simulink model "Sensors"  (R2026a)
settings: Solver=FixedStepAuto
values from neighbouring files (symbols this model uses):
  SNS = loadSensorParameters()    [ch7_main.m]    (also in loadSensorParameters.m = struct())
undefined symbols (not defined in the file or in its folder): DiscIntNeverNeededParam, MAV, SIM
libraries: simulink x8
settings Model: Creator=emrec  LastModifiedBy=emrec

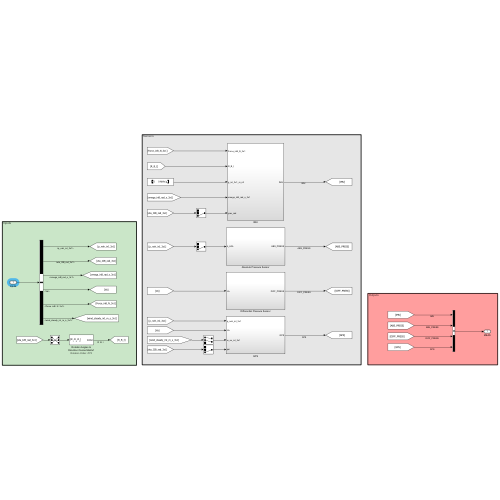
[thumbnail: Simulink's stored preview of the top-level diagram]
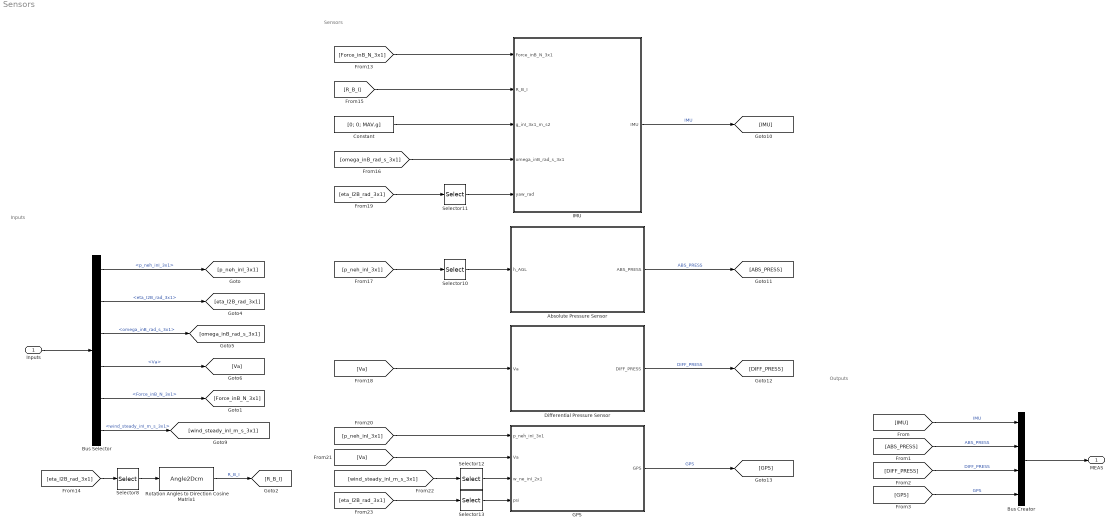
== system Sensors ==
  note: Outputs
  note: Sensors
  note: Inputs
  Inputs : Inport  OutDataTypeStr=Bus: SensorsInputsBus
  Absolute Pressure Sensor : Subsystem
  Bus Creator : BusCreator  Inputs=4
  Bus Selector : BusSelector  OutputSignals=p_neh_inI_3x1,eta_I2B_rad_3x1,omega_inB_rad_s_3x1,Va,Force_inB_N_3x1,wind_steady_inI_m_s_3x1
  Constant : Constant  Value=[0; 0; MAV.g]
  Differential Pressure Sensor : Subsystem
  GPS : Subsystem
  IMU : Subsystem
  Rotation Angles to Direction Cosine Matrix1 : Angle2Dcm
      settings: AttributesFormatString=Rotation Order: %<rotationOrder>
  Selector10 : Selector  InputPortWidth=3  IndexOptions=Index vector (dialog)  Indices=[3]  OutputSizes=1
  Selector11 : Selector  InputPortWidth=3  IndexOptions=Index vector (dialog)  Indices=[3]  OutputSizes=1
  Selector12 : Selector  InputPortWidth=3  IndexOptions=Index vector (dialog)  Indices=[1 2]  OutputSizes=1
  Selector13 : Selector  InputPortWidth=3  IndexOptions=Index vector (dialog)  Indices=[3]  OutputSizes=1
  Selector8 : Selector  InputPortWidth=3  IndexOptions=Index vector (dialog)  Indices=[3 2 1]  OutputSizes=1
  MEAS : Outport  OutDataTypeStr=Bus: SensorsMeasBus
  wires:
  Absolute Pressure Sensor/1(ABS_PRESS) -> [ABS_PRESS]  "ABS_PRESS"
  Differential Pressure Sensor/1(DIFF_PRESS) -> [DIFF_PRESS]  "DIFF_PRESS"
  Rotation Angles to Direction Cosine Matrix1/1 -> [R_B_I]  "R_B_I"
  Bus Selector/6 -> [wind_steady_inI_m_s_3x1]  "<wind_steady_inI_m_s_3x1>"
  Selector8/1 -> Rotation Angles to Direction Cosine Matrix1/1
  Bus Selector/1 -> [p_neh_inI_3x1]  "<p_neh_inI_3x1>"
  Bus Selector/4 -> [Va]  "<Va>"
  Bus Selector/3 -> [omega_inB_rad_s_3x1]  "<omega_inB_rad_s_3x1>"
  Bus Selector/5 -> [Force_inB_N_3x1]  "<Force_inB_N_3x1>"
  [eta_I2B_rad_3x1] -> Selector8/1
  Inputs/1 -> Bus Selector/1
  Bus Selector/2 -> [eta_I2B_rad_3x1]  "<eta_I2B_rad_3x1>"
  [R_B_I] -> IMU/2(R_B_I)
  [Force_inB_N_3x1] -> IMU/1(Force_inB_N_3x1)
  Constant/1 -> IMU/3(g_inI_3x1_m_s2)
  [omega_inB_rad_s_3x1] -> IMU/4(omega_inB_rad_s_3x1)
  Selector11/1 -> IMU/5(yaw_rad)
  [eta_I2B_rad_3x1] -> Selector11/1
  Selector10/1 -> Absolute Pressure Sensor/1(h_AGL)
  [p_neh_inI_3x1] -> Selector10/1
  [Va] -> Differential Pressure Sensor/1(Va)
  [eta_I2B_rad_3x1] -> Selector13/1
  [wind_steady_inI_m_s_3x1] -> Selector12/1
  [Va] -> GPS/2(Va)
  [p_neh_inI_3x1] -> GPS/1(p_neh_inI_3x1)
  Selector12/1 -> GPS/3(w_ne_inI_2x1)
  Selector13/1 -> GPS/4(psi)
  GPS/1(GPS) -> [GPS]  "GPS"
  IMU/1(IMU) -> [IMU]  "IMU"
  [IMU] -> Bus Creator/1  "IMU"
  [ABS_PRESS] -> Bus Creator/2  "ABS_PRESS"
  [DIFF_PRESS] -> Bus Creator/3  "DIFF_PRESS"
  [GPS] -> Bus Creator/4  "GPS"
  Bus Creator/1 -> MEAS/1

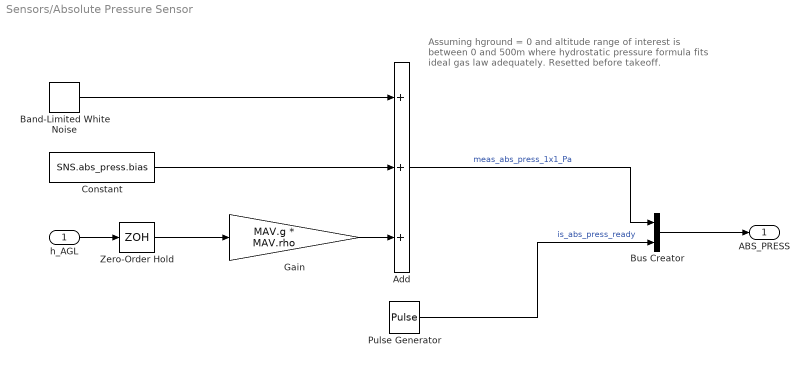
== system Sensors/Absolute Pressure Sensor ==
  note: Assuming hground = 0 and altitude range of interest is
      | between 0 and 500m where hydrostatic pressure formula
      | fits ideal gas law adequately.
      |
      | Resetted before takeoff.
  h_AGL : Inport
  Add : Sum  Inputs=+++
  Band-Limited White Noise : simulink/Sources/Band-Limited White Noise  Cov=[SNS.abs_press.var] * SNS.abs_press.Ts  Ts=SNS.abs_press.Ts  seed=[SNS.abs_press.seed]
  Bus Creator : BusCreator  Inputs=2
  Constant : Constant  Value=SNS.abs_press.bias
  Gain : Gain  Gain=MAV.g * MAV.rho
  Pulse Generator : DiscretePulseGenerator  Period=SNS.abs_press.Ts / SIM.FixedStepSize  SampleTime=SIM.FixedStepSize
  Zero-Order Hold : ZeroOrderHold  SampleTime=SNS.abs_press.Ts
  ABS_PRESS : Outport
  wires:
  Band-Limited White Noise/1 -> Add/1
  Constant/1 -> Add/2
  Gain/1 -> Add/3
  h_AGL/1 -> Zero-Order Hold/1
  Zero-Order Hold/1 -> Gain/1
  Pulse Generator/1 -> Bus Creator/2  "is_abs_press_ready"
  Add/1 -> Bus Creator/1  "meas_abs_press_1x1_Pa"
  Bus Creator/1 -> ABS_PRESS/1

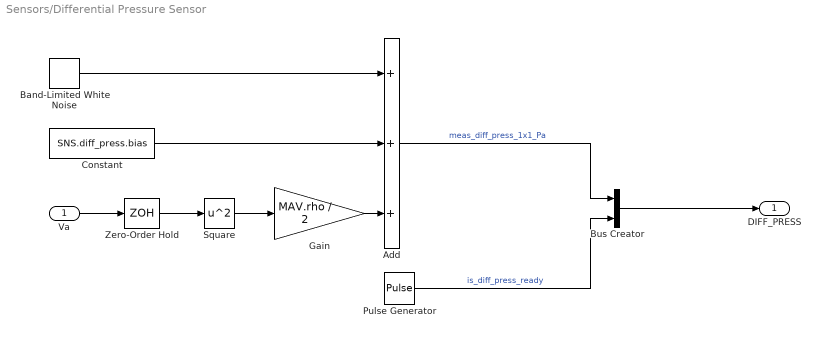
== system Sensors/Differential Pressure Sensor ==
  Va : Inport
  Add : Sum  Inputs=+++
  Band-Limited White Noise : simulink/Sources/Band-Limited White Noise  Cov=[SNS.diff_press.var] * SNS.diff_press.Ts  Ts=SNS.diff_press.Ts  seed=[SNS.diff_press.seed]
  Bus Creator : BusCreator  Inputs=2
  Constant : Constant  Value=SNS.diff_press.bias
  Gain : Gain  Gain=MAV.rho / 2
  Pulse Generator : DiscretePulseGenerator  Period=SNS.diff_press.Ts / SIM.FixedStepSize  SampleTime=SIM.FixedStepSize
  Square : Math  Operator=square
  Zero-Order Hold : ZeroOrderHold  SampleTime=SNS.diff_press.Ts
  DIFF_PRESS : Outport
  wires:
  Square/1 -> Gain/1
  Va/1 -> Zero-Order Hold/1
  Gain/1 -> Add/3
  Constant/1 -> Add/2
  Band-Limited White Noise/1 -> Add/1
  Zero-Order Hold/1 -> Square/1
  Pulse Generator/1 -> Bus Creator/2  "is_diff_press_ready"
  Add/1 -> Bus Creator/1  "meas_diff_press_1x1_Pa"
  Bus Creator/1 -> DIFF_PRESS/1

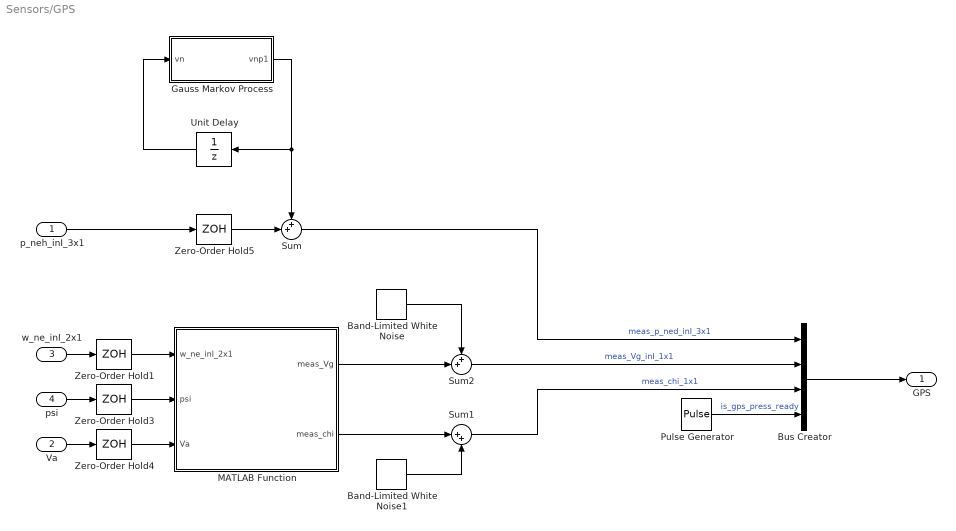
== system Sensors/GPS ==
  p_neh_inI_3x1 : Inport
  Va : Inport  Port=2
  w_ne_inI_2x1 : Inport  Port=3
  psi : Inport  Port=4
  Band-Limited White Noise : simulink/Sources/Band-Limited White Noise  Cov=[SNS.gps.var_vg] * SNS.gps.Ts  Ts=SNS.gps.Ts  seed=[SNS.gps.seed_vg]
  Band-Limited White Noise1 : simulink/Sources/Band-Limited White Noise  Cov=[SNS.gps.var_chi] * SNS.gps.Ts  Ts=SNS.gps.Ts  seed=[SNS.gps.seed_chi]
  Bus Creator : BusCreator  Inputs=4
  Gauss Markov Process : Subsystem
  MATLAB Function : MATLAB Function  TreatAsAtomicUnit=on
  Pulse Generator : DiscretePulseGenerator  Period=SNS.gps.Ts / SIM.FixedStepSize  SampleTime=SIM.FixedStepSize
  Sum : Sum  Inputs=++|
  Sum1 : Sum  Inputs=|++
  Sum2 : Sum  Inputs=++|
  Unit Delay : UnitDelay  InitialCondition=SNS.gps.v0  SampleTime=SNS.gps.Ts
  Zero-Order Hold{1,3..5} (4 alike) : ZeroOrderHold  SampleTime=SNS.gps.Ts
  GPS : Outport
  wires:
  Band-Limited White Noise/1 -> Sum2/1
  MATLAB Function/1(meas_Vg) -> Sum2/2
  Band-Limited White Noise1/1 -> Sum1/2
  MATLAB Function/2(meas_chi) -> Sum1/1
  psi/1 -> Zero-Order Hold3/1
  w_ne_inI_2x1/1 -> Zero-Order Hold1/1
  Va/1 -> Zero-Order Hold4/1
  p_neh_inI_3x1/1 -> Zero-Order Hold5/1
  Unit Delay/1 -> Gauss Markov Process/1(vn)
  Gauss Markov Process/1(vnp1) -> Unit Delay/1, Sum/1
  Zero-Order Hold1/1 -> MATLAB Function/1(w_ne_inI_2x1)
  Zero-Order Hold3/1 -> MATLAB Function/2(psi)
  Zero-Order Hold4/1 -> MATLAB Function/3(Va)
  Zero-Order Hold5/1 -> Sum/2
  Sum/1 -> Bus Creator/1  "meas_p_ned_inI_3x1"
  Sum2/1 -> Bus Creator/2  "meas_Vg_inI_1x1"
  Sum1/1 -> Bus Creator/3  "meas_chi_1x1"
  Pulse Generator/1 -> Bus Creator/4  "is_gps_press_ready"
  Bus Creator/1 -> GPS/1

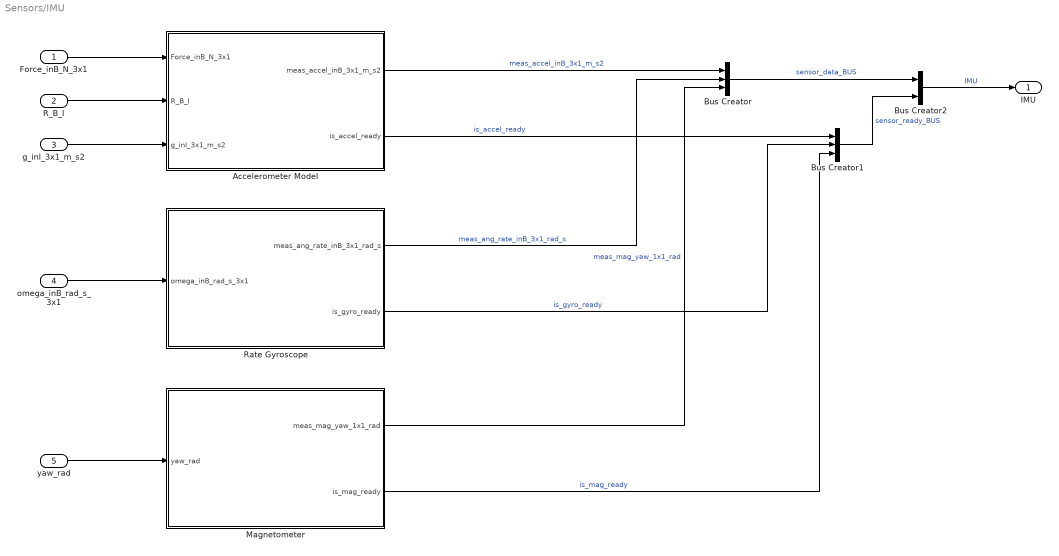
== system Sensors/IMU ==
  Force_inB_N_3x1 : Inport
  R_B_I : Inport  Port=2
  g_inI_3x1_m_s2 : Inport  Port=3
  omega_inB_rad_s_3x1 : Inport  Port=4
  yaw_rad : Inport  Port=5
  Accelerometer Model : Subsystem
  Bus Creator : BusCreator  Inputs=3
  Bus Creator1 : BusCreator  Inputs=3
  Bus Creator2 : BusCreator  Inputs=2
  Magnetometer : Subsystem
  Rate Gyroscope : Subsystem  SystemSampleTime=1 / SNS.gyro.SamplingRate
  IMU : Outport
  wires:
  Magnetometer/1("meas_mag_yaw_1x1_rad ") -> Bus Creator/3  "meas_mag_yaw_1x1_rad"
  Accelerometer Model/1(meas_accel_inB_3x1_m_s2) -> Bus Creator/1  "meas_accel_inB_3x1_m_s2"
  Rate Gyroscope/1(meas_ang_rate_inB_3x1_rad_s) -> Bus Creator/2  "meas_ang_rate_inB_3x1_rad_s"
  Force_inB_N_3x1/1 -> Accelerometer Model/1(Force_inB_N_3x1)
  R_B_I/1 -> Accelerometer Model/2(R_B_I)
  g_inI_3x1_m_s2/1 -> Accelerometer Model/3(g_inI_3x1_m_s2)
  omega_inB_rad_s_3x1/1 -> Rate Gyroscope/1(omega_inB_rad_s_3x1)
  yaw_rad/1 -> Magnetometer/1(yaw_rad)
  Rate Gyroscope/2(is_gyro_ready) -> Bus Creator1/2  "is_gyro_ready"
  Accelerometer Model/2(is_accel_ready) -> Bus Creator1/1  "is_accel_ready"
  Magnetometer/2(is_mag_ready) -> Bus Creator1/3  "is_mag_ready"
  Bus Creator/1 -> Bus Creator2/1  "sensor_data_BUS"
  Bus Creator1/1 -> Bus Creator2/2  "sensor_ready_BUS"
  Bus Creator2/1 -> IMU/1  "IMU"

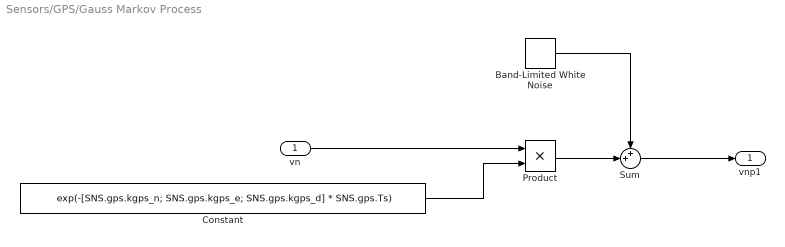
== system Sensors/GPS/Gauss Markov Process ==
  vn : Inport
  Band-Limited White Noise : simulink/Sources/Band-Limited White Noise  Cov=[SNS.gps.var_n; SNS.gps.var_e; SNS.gps.var_d] * SNS.gps.Ts  Ts=SNS.gps.Ts  seed=[SNS.gps.seed_n; SNS.gps.seed_e; SNS.gps.seed_d]
  Constant : Constant  Value=exp(-[SNS.gps.kgps_n; SNS.gps.kgps_e; SNS.gps.kgps_d] * SNS.gps.Ts)
  Product : Product
  Sum : Sum  Inputs=++|
  vnp1 : Outport
  wires:
  Sum/1 -> vnp1/1
  Band-Limited White Noise/1 -> Sum/1
  Product/1 -> Sum/2
  Constant/1 -> Product/2
  vn/1 -> Product/1

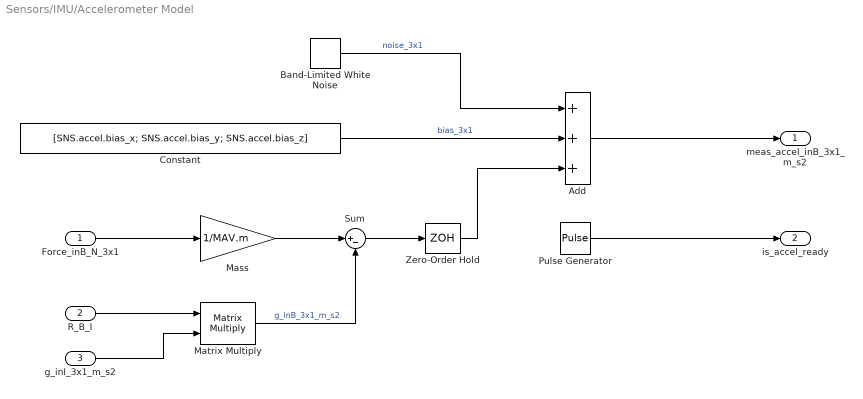
== system Sensors/IMU/Accelerometer Model ==
  Force_inB_N_3x1 : Inport
  R_B_I : Inport  Port=2
  g_inI_3x1_m_s2 : Inport  Port=3
  Add : Sum  Inputs=+++
  Band-Limited White Noise : simulink/Sources/Band-Limited White Noise  Cov=[SNS.accel.var_x; SNS.accel.var_y; SNS.accel.var_z] * SNS.accel.Ts  Ts=SNS.accel.Ts  seed=[SNS.accel.seed_x; SNS.accel.seed_y; SNS.accel.seed_z]
  Constant : Constant  Value=[SNS.accel.bias_x; SNS.accel.bias_y; SNS.accel.bias_z]
  Mass : Gain  Gain=1/MAV.m
  Matrix Multiply : Product  Multiplication=Matrix(*)
  Pulse Generator : DiscretePulseGenerator  Period=SNS.accel.Ts / SIM.FixedStepSize  SampleTime=SIM.FixedStepSize
  Sum : Sum  Inputs=|+-
  Zero-Order Hold : ZeroOrderHold  SampleTime=SNS.accel.Ts
  meas_accel_inB_3x1_m_s2 : Outport
  is_accel_ready : Outport  Port=2
  wires:
  Sum/1 -> Zero-Order Hold/1
  Band-Limited White Noise/1 -> Add/1  "noise_3x1"
  Constant/1 -> Add/2  "bias_3x1"
  Mass/1 -> Sum/1
  Force_inB_N_3x1/1 -> Mass/1
  Matrix Multiply/1 -> Sum/2  "g_inB_3x1_m_s2"
  g_inI_3x1_m_s2/1 -> Matrix Multiply/2
  R_B_I/1 -> Matrix Multiply/1
  Zero-Order Hold/1 -> Add/3
  Add/1 -> meas_accel_inB_3x1_m_s2/1
  Pulse Generator/1 -> is_accel_ready/1

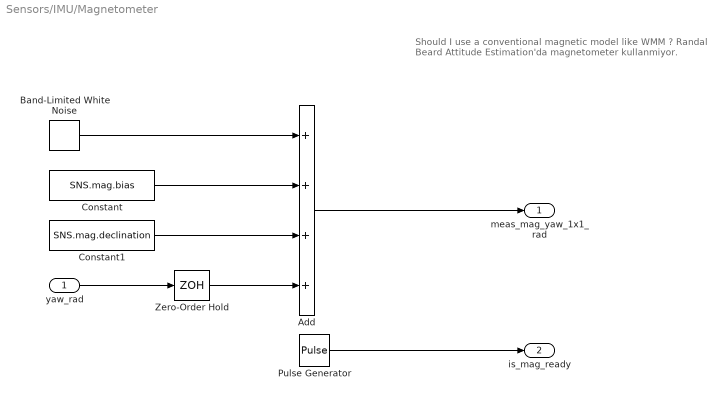
== system Sensors/IMU/Magnetometer ==
  note: Should I use a conventional magnetic model like WMM ?
      |
      |
      | Randal Beard Attitude Estimation'da magnetometer kullanmiyor.
  yaw_rad : Inport
  Add : Sum  Inputs=++++
  Band-Limited White Noise : simulink/Sources/Band-Limited White Noise  Cov=[SNS.mag.var] * SNS.mag.Ts  Ts=SNS.mag.Ts  seed=[SNS.mag.seed]
  Constant : Constant  Value=SNS.mag.bias
  Constant1 : Constant  Value=SNS.mag.declination
  Pulse Generator : DiscretePulseGenerator  Period=SNS.mag.Ts / SIM.FixedStepSize  SampleTime=SIM.FixedStepSize
  Zero-Order Hold : ZeroOrderHold  SampleTime=SNS.mag.Ts
  "meas_mag_yaw_1x1_rad " : Outport
  is_mag_ready : Outport  Port=2
  wires:
  Constant1/1 -> Add/3
  Band-Limited White Noise/1 -> Add/1
  Constant/1 -> Add/2
  yaw_rad/1 -> Zero-Order Hold/1
  Zero-Order Hold/1 -> Add/4
  Add/1 -> "meas_mag_yaw_1x1_rad "/1
  Pulse Generator/1 -> is_mag_ready/1

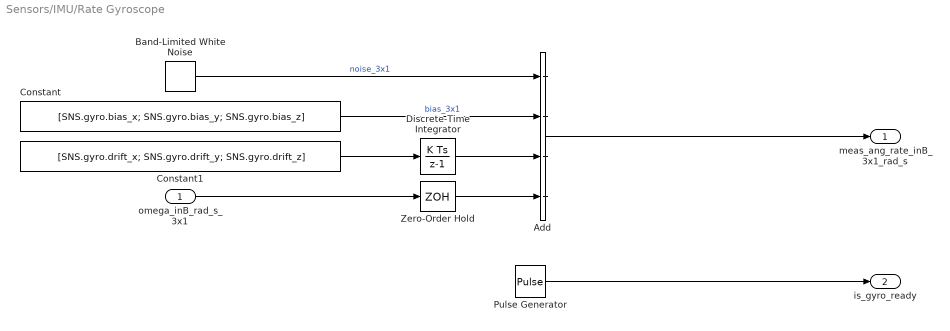
== system Sensors/IMU/Rate Gyroscope ==
  omega_inB_rad_s_3x1 : Inport
  Add : Sum  Inputs=++++
  Band-Limited White Noise : simulink/Sources/Band-Limited White Noise  Cov=[SNS.gyro.var_x; SNS.gyro.var_y; SNS.gyro.var_z] * SNS.gyro.Ts  Ts=SNS.gyro.Ts  seed=[SNS.gyro.seed_x; SNS.gyro.seed_y; SNS.gyro.seed_z]
  Constant : Constant  Value=[SNS.gyro.bias_x; SNS.gyro.bias_y; SNS.gyro.bias_z]
  Constant1 : Constant  Value=[SNS.gyro.drift_x; SNS.gyro.drift_y; SNS.gyro.drift_z]
  Discrete-Time Integrator : DiscreteIntegrator  SampleTime=SNS.gyro.Ts  ICPrevOutput=DiscIntNeverNeededParam  ICPrevScaledInput=DiscIntNeverNeededParam
  Pulse Generator : DiscretePulseGenerator  Period=SNS.gyro.Ts / SIM.FixedStepSize  SampleTime=SIM.FixedStepSize
  Zero-Order Hold : ZeroOrderHold  SampleTime=SNS.gyro.Ts
  meas_ang_rate_inB_3x1_rad_s : Outport
  is_gyro_ready : Outport  Port=2
  wires:
  omega_inB_rad_s_3x1/1 -> Zero-Order Hold/1
  Discrete-Time Integrator/1 -> Add/3
  Constant1/1 -> Discrete-Time Integrator/1
  Constant/1 -> Add/2  "bias_3x1"
  Band-Limited White Noise/1 -> Add/1  "noise_3x1"
  Add/1 -> meas_ang_rate_inB_3x1_rad_s/1
  Zero-Order Hold/1 -> Add/4
  Pulse Generator/1 -> is_gyro_ready/1

== matlab function Sensors/GPS/MATLAB Function ==
  data: w_ne_inI_2x1 input; psi input; Va input; meas_Vg output; meas_chi output
function [meas_Vg, meas_chi] = gps_Vg_chi(w_ne_inI_2x1, psi, Va)
    Vn = Va * cos(psi) + w_ne_inI_2x1(1);
    Ve = Va * sin(psi) + w_ne_inI_2x1(2);

    meas_Vg = sqrt(Vn^2 + Ve^2);

    meas_chi = atan2(Ve, Vn);
end
